simulink library "ASEToolBox"  (R2025b)
settings: Solver=ode45  StartTime=0.0  StopTime=10.0  RelTol=1e-3  EnableMultiTasking=on
values from neighbouring files (symbols this model uses):
  dt = get_param(gcbh, 'g_output_datatype')    [maskSysComCallbacks_Receive.m]    (also in maskSysComCallbacks_Send.m = get_param(gcbh, 'g_input_datatype'))
undefined symbols (not defined in the file or in its folder): dCx, dCy, dCz, DiscIntNeverNeededParam, Discrete, dmassX, dmassY, dmassZ, dMx, dMy, dMz, dp, dp0, dp1, dp2, dp3, dspblkCoreblockFVToolHelper, gcbh, lmd_high, lmd_low, magnitude, Newton, p0, p1, p2, p3, p4, phi0, phi000, phi1, phi2, phi3, phi4, r1, r2, r3, r4, Raphson, theta0, theta1, theta2, theta3, theta4, Time, u0, u1, u2, u3, v0, v0_max, v0_min, v1, v111, v2, v222, v3, v333, v4, W1, w1 ... (+4)
libraries: simulink x38, etargetslib x28, simulink_extras x5, slpidlib x2, ctrlSharedLib x2, aerolibatmos2 x1, aerolibconvert2 x1, aerolibtransform2 x1, sharedtransform x1, dspstat3 x1, dspsolvers x1
(part 5 of 6)

== system ASEToolBox/Subsystem/GNC_EKF/GPS_Data_Process/heading_GPS ==
  Vned : Inport
  Atan2 : Trigonometry  Operator=atan2
  Compare To Constant : simulink/Logic and Bit Operations/Compare To Constant  relop=>  const=0.8  OutDataTypeStr=boolean
  Data Type Conversion : DataTypeConversion  OutDataTypeStr=double  SaturateOnIntegerOverflow=off  RndMeth=Floor
  Math Function : Math  Operator=magnitude^2  SignedPower=on
  Moving Average1 : dspstat3/Moving Average  Commented=on  Method=Sliding window  ForgettingFactorPort=off  SpecifyWindowLength=on  WindowLength=10  OverlapLength=9  AllowArbitraryInputLength=off  ForgettingFactor=0.9  SimulateUsing=Code generation
  Rate Transition : RateTransition  OutPortSampleTime=1
  Scope : Scope  NumInputPorts=2
      settings: ActiveDisplayYMinimum=-3.92587  ActiveDisplayYMaximum=3.91959  DataLoggingVariableName=ScopeData11
  Scope1 : Scope
      settings: ActiveDisplayYMinimum=-0.125  ActiveDisplayYMaximum=1.125  DataLoggingVariableName=ScopeData14
  Selector2 : Selector  InputPortWidth=3  IndexOptions=Index vector (dialog)  Indices=[2]  OutputSizes=1
  Selector3 : Selector  InputPortWidth=3  IndexOptions=Index vector (dialog)  Indices=[1]  OutputSizes=1
  Selector4 : Selector  InputPortWidth=3  IndexOptions=Index vector (dialog)  Indices=[1 2]  OutputSizes=1
  Sqrt : Sqrt
  Sum of Elements : Sum  Inputs=+
  heading_GPS_rad : Outport
  heading_GPS_valid : Outport  Port=2
  wires:
  Selector2/1 -> Atan2/1
  Math Function/1 -> Sum of Elements/1
  Vned/1 -> Selector2/1, Selector4/1, Selector3/1
  Selector3/1 -> Atan2/2
  Sum of Elements/1 -> Sqrt/1
  Selector4/1 -> Math Function/1
  Sqrt/1 -> Data Type Conversion/1
  Compare To Constant/1 -> Scope1/1, heading_GPS_valid/1
  Rate Transition/1 -> Scope/1, Scope/2, heading_GPS_rad/1
  Atan2/1 -> Rate Transition/1
  Data Type Conversion/1 -> Compare To Constant/1

== system ASEToolBox/Subsystem/GNC_EKF/Translation_estimate/Subsystem ==
  vxy : Inport
  pxy_GPS : Inport  Port=2
  GPSv_enable : Inport  Port=3
  QGC_init : Inport  Port=4
  DOP : Inport  Port=5
  Add : Sum  Inputs=+-
  Add1 : Sum  Inputs=++-
  Compare To Constant : simulink/Logic and Bit Operations/Compare To Constant  relop=<=  const=3  OutDataTypeStr=boolean
  Delay : Delay  DelayLength=1  InitialCondition=[0;0;]  ExternalReset=Rising
      settings: InputPortMap=u0,r5
  Detect Change : simulink/Logic and Bit Operations/Detect Change  vinit=0  OutDataTypeStr=boolean
  Gain : Gain  Gain=0.002
  Kalman Filter : ctrlSharedLib/Kalman Filter  TimeDomain=Discrete-Time  UseCurrentEstimator=on  ModelSource=Individual A, B, C, D matrices  ModelSourceVariable=ss(0.95,1,1,0,1)  A=[0.1,0;0,0.1]  B=eye(2)  C=eye(2)  D=0  NumberOfStates=1  NumberOfInputs=1  NumberOfOutputs=1  InitialEstimateSource=Dialog  X0=0  P0=10  UseK=off  UseGH=off  NumberOfProcessNoiseInputs=1  G=1  TimeInvariantG=on  H=0  TimeInvariantH=on  Q=diag([0.1;0.1])  TimeInvariantQ=on  R=diag([0.8;0.8])  TimeInvariantR=on  N=0  TimeInvariantN=on  AddInputPort=off  AddEnablePort=on  ExternalReset=Rising  OutputEstimatedY=off  OutputP=off  Ts=-1
  Logical Operator : Logic  AllPortsSameDT=off  OutDataTypeStr=boolean
  Memory : Memory
  Product : Product  OutDataTypeStr=double
  QGC_init1 : InportShadow  Port=4
  Rate Transition1 : RateTransition  OutPortSampleTime=0.002
  Rate Transition2 : RateTransition  OutPortSampleTime=0.002
  Rate Transition3 : RateTransition  OutPortSampleTime=0.002
  Scope7 : Scope
      settings: ActiveDisplayYMinimum=-0.125  ActiveDisplayYMaximum=1.125
  Selector : Selector  InputPortWidth=2  IndexOptions=Index vector (dialog)  Indices=[1]  OutputSizes=1
  pxy_est : Outport
  wires:
  Gain/1 -> Add1/1
  Delay/1 -> Add1/2
  Kalman Filter/1 -> Product/1
  pxy_GPS/1 -> Selector/1, Add/2
  Selector/1 -> Detect Change/1
  Product/1 -> Memory/1
  Logical Operator/1 -> Product/2, Rate Transition2/1
  Rate Transition2/1 -> Scope7/1, Kalman Filter/2
  Rate Transition1/1 -> Kalman Filter/1
  Memory/1 -> Add1/3
  Add/1 -> Rate Transition1/1
  vxy/1 -> Gain/1
  Add1/1 -> Add/1, Delay/1, pxy_est/1
  QGC_init/1 -> Rate Transition3/1
  Rate Transition3/1 -> Kalman Filter/3
  DOP/1 -> Compare To Constant/1
  Compare To Constant/1 -> Logical Operator/2
  QGC_init1/1 -> Delay/2
  GPSv_enable/1 -> Logical Operator/1

== system ASEToolBox/Subsystem/GNC_EKF/Translation_estimate/Subsystem2 ==
  axy : Inport
  vxy_GPS : Inport  Port=2
  QGC_init : Inport  Port=3
  DOP : Inport  Port=4
  Add : Sum  Inputs=+-
  Add1 : Sum  Inputs=++-
  Compare To Constant : simulink/Logic and Bit Operations/Compare To Constant  relop=<=  const=3  OutDataTypeStr=boolean
  Delay : Delay  DelayLength=1  ExternalReset=Rising
      settings: InputPortMap=u0,r5
  Detect Change : simulink/Logic and Bit Operations/Detect Change  vinit=0  OutDataTypeStr=boolean
  Gain : Gain  Gain=0.002
  Kalman Filter : ctrlSharedLib/Kalman Filter  TimeDomain=Discrete-Time  UseCurrentEstimator=on  ModelSource=Individual A, B, C, D matrices  ModelSourceVariable=ss(0.95,1,1,0,1)  A=[0.6,0;0,0.6]  B=eye(2)  C=eye(2)  D=0  NumberOfStates=1  NumberOfInputs=1  NumberOfOutputs=1  InitialEstimateSource=Dialog  X0=0  P0=10  UseK=off  UseGH=off  NumberOfProcessNoiseInputs=1  G=1  TimeInvariantG=on  H=0  TimeInvariantH=on  Q=diag([0.1;0.1])  TimeInvariantQ=on  R=diag([0.6;0.6])  TimeInvariantR=on  N=0  TimeInvariantN=on  AddInputPort=off  AddEnablePort=on  ExternalReset=Rising  OutputEstimatedY=off  OutputP=off  Ts=-1
  Logical Operator : Logic  AllPortsSameDT=off  OutDataTypeStr=boolean
  Memory : Memory
  Product : Product  OutDataTypeStr=double
  Rate Transition1 : RateTransition  OutPortSampleTime=0.002
  Rate Transition2 : RateTransition  OutPortSampleTime=0.002
  Rate Transition3 : RateTransition  OutPortSampleTime=0.002
  Scope : Scope  NumInputPorts=2
      settings: ActiveDisplayYMinimum=-13.99764  ActiveDisplayYMaximum=33.23237
  Scope7 : Scope
      settings: ActiveDisplayYMinimum=-0.125  ActiveDisplayYMaximum=1.125
  Selector : Selector  InputPortWidth=2  IndexOptions=Index vector (dialog)  Indices=[1]  OutputSizes=1
  vxy_est : Outport
  GPSv_enable : Outport  Port=2
  wires:
  Compare To Constant/1 -> Logical Operator/2
  DOP/1 -> Compare To Constant/1
  Detect Change/1 -> Logical Operator/1
  Rate Transition3/1 -> Kalman Filter/3
  QGC_init/1 -> Delay/2, Rate Transition3/1
  Add1/1 -> Delay/1, vxy_est/1, Scope/1, Add/1
  Add/1 -> Rate Transition1/1
  Memory/1 -> Add1/3
  Rate Transition1/1 -> Kalman Filter/1
  Rate Transition2/1 -> Scope7/1, Kalman Filter/2
  Logical Operator/1 -> GPSv_enable/1, Rate Transition2/1, Product/2
  Product/1 -> Memory/1
  Selector/1 -> Detect Change/1
  vxy_GPS/1 -> Selector/1, Add/2, Scope/2
  Kalman Filter/1 -> Product/1
  Gain/1 -> Add1/1
  axy/1 -> Gain/1
  Delay/1 -> Add1/2

== system ASEToolBox/Subsystem/GNC_EKF/Translation_estimate/V_Horizontal_estimation1 ==
  note: 0530改：
      | 加入GPStype限制
  An : Inport
  vn_gps : Inport  Port=2
  ve_gps : Inport  Port=3
  fixtype_gps : Inport  Port=4
  QGC_init : Inport  Port=5
  Add : Sum  Inputs=+-
  Compare To Constant : simulink/Logic and Bit Operations/Compare To Constant  relop=>=  const=3  OutDataTypeStr=boolean
  Delay : Delay  DelayLength=1
  Detect Change : simulink/Logic and Bit Operations/Detect Change  vinit=0  OutDataTypeStr=boolean
  Integrator_V_Horizontal : Subsystem
  Logical Operator : Logic  AllPortsSameDT=off  OutDataTypeStr=boolean
  Mux : Mux  Inputs=2
  Rxy_kalman filter1 : Subsystem  mask{F=diag([-0.1,-0.1,-0.002,-0.002]), H=[1,0,-1,0;0,1,0,-1], Q=diag([1,1,0.1,0.1]), R=diag([0.001,0.001]), P0=diag([0.8,0.8,0.2,0.2])}
      mask prompts: F "状态转移矩阵：F"; H "观测转移矩阵：H"; Q "预测噪声协方差矩阵：Q"; R "量测噪声协方差矩阵：R"; P0 "初始协方差矩阵：P0"
      mask DialogControl DescTextVar Prompt: Kalman Filter
  Scope : Scope  NumInputPorts=2
      settings: ActiveDisplayYMinimum=-0.21744  ActiveDisplayYMaximum=0.36084  DataLoggingVariableName=ScopeData16
  Scope1 : Scope
      settings: ActiveDisplayYMinimum=0.9  ActiveDisplayYMaximum=1.1
  Selector : Selector  InputPortWidth=4  IndexOptions=Index vector (dialog)  Indices=[1 2]  OutputSizes=1
  vxy_estimout : Outport
  GPS_v_enable : Outport  Port=2
  wires:
  QGC_init/1 -> Integrator_V_Horizontal/3(QGC_init)
  Delay/1 -> Selector/1, Rxy_kalman filter1/1(X)
  Selector/1 -> Integrator_V_Horizontal/2(dv)
  vn_gps/1 -> Integrator_V_Horizontal/4(vn_gps), Mux/1, Detect Change/1
  Mux/1 -> Scope/2, Add/2
  ve_gps/1 -> Integrator_V_Horizontal/5(ve_gps), Mux/2
  Rxy_kalman filter1/1(XOut) -> Delay/1
  Integrator_V_Horizontal/1(V_n&e) -> Add/1, vxy_estimout/1, Scope/1
  Add/1 -> Rxy_kalman filter1/2(Z)
  An/1 -> Integrator_V_Horizontal/1(An)
  fixtype_gps/1 -> Compare To Constant/1
  Detect Change/1 -> Logical Operator/1
  Compare To Constant/1 -> Logical Operator/2, Scope1/1, GPS_v_enable/1, Rxy_kalman filter1/3(Enable), Integrator_V_Horizontal/6(GPSenable)

== system ASEToolBox/Subsystem/GNC_EKF/Translation_estimate/translate to N ==
  Cbn : Inport
  accl_ned : Inport  Port=2
  Product : Product  Multiplication=Matrix(*)
  Selector : Selector  InputPortWidth=3  IndexOptions=Index vector (dialog)  Indices=[1 2]  OutputSizes=1
  accel_Horizontal_predict : Outport
  wires:
  Selector/1 -> accel_Horizontal_predict/1
  Product/1 -> Selector/1
  Cbn/1 -> Product/1
  accl_ned/1 -> Product/2

== system ASEToolBox/Aerocraft Model/ACE Equation of 6DOF's Motion/ACE Centroid Motion/231 Motion Subsystem/Deal with zero1 ==
  In1 : Inport
  Constant : Constant  Value=0
  Constant1 : Constant  Value=0.000001
  Relational Operator : RelationalOperator  Operator=~=
  Switch : Switch  Threshold=0.0001
  Out1 : Outport
  wires:
  In1/1 -> Relational Operator/1, Switch/1
  Switch/1 -> Out1/1
  Constant1/1 -> Switch/3
  Relational Operator/1 -> Switch/2
  Constant/1 -> Relational Operator/2

== system ASEToolBox/Aerocraft Model/ACE Equation of 6DOF's Motion/ACE Centroid Motion/231 Motion Subsystem/Deal with zero2 ==
  In1 : Inport
  Constant : Constant  Value=0
  Constant1 : Constant  Value=0.000001
  Relational Operator : RelationalOperator  Operator=~=
  Switch : Switch  Threshold=0.0001
  Out1 : Outport
  wires:
  Constant/1 -> Relational Operator/2
  Relational Operator/1 -> Switch/2
  Constant1/1 -> Switch/3
  Switch/1 -> Out1/1
  In1/1 -> Switch/1, Relational Operator/1

== system ASEToolBox/Aerocraft Model/ACE Equation of 6DOF's Motion/ACE Centroid Motion/231 Motion Subsystem/Deal with zero3 ==
  In1 : Inport
  Constant : Constant  Value=0
  Constant1 : Constant  Value=0.000001
  Relational Operator : RelationalOperator  Operator=~=
  Switch : Switch  Threshold=0.0001
  Out1 : Outport
  wires:
  Constant/1 -> Relational Operator/2
  Relational Operator/1 -> Switch/2
  Constant1/1 -> Switch/3
  Switch/1 -> Out1/1
  In1/1 -> Switch/1, Relational Operator/1

== system ASEToolBox/Aerocraft Model/ACE Equation of 6DOF's Motion/ACE Rotation Motion/Attitude Dynamic /Omega_Tx1 Subsystem ==
  note: d( w_x ) = [M_x + (I_y-I_z)*w_y*w_z)] / I_x
      | .
  note: rad/s
  Wxyz : Inport
  Ixyz : Inport  Port=2
  Mxyz : Inport  Port=3
  Deal with zero : Subsystem
  Demux6 : Demux  Outputs=3
  Discrete-Time Integrator : DiscreteIntegrator  SampleTime=-1  ICPrevOutput=DiscIntNeverNeededParam  ICPrevScaledInput=DiscIntNeverNeededParam
  Integrator1 : Integrator  Commented=on
  Product4 : Product  Inputs=***  InputSameDT=on  SaturateOnIntegerOverflow=on  OutDataTypeStr=Inherit: Same as first input
  Product6 : Product  Inputs=/*  InputSameDT=on  SaturateOnIntegerOverflow=on  OutDataTypeStr=Inherit: Same as first input
  Selector1 : Selector  InputPortWidth=3  IndexOptions=Index vector (dialog)  Indices=2  OutputSizes=1
  Selector2 : Selector  InputPortWidth=3  IndexOptions=Index vector (dialog)  Indices=1  OutputSizes=1
  Selector3 : Selector  InputPortWidth=3  IndexOptions=Index vector (dialog)  Indices=3  OutputSizes=1
  Sum1 : Sum  Inputs=+-  InputSameDT=on  SaturateOnIntegerOverflow=on  OutDataTypeStr=Inherit: Same as first input
  Sum6 : Sum  InputSameDT=on  SaturateOnIntegerOverflow=on  OutDataTypeStr=Inherit: Same as first input
  Wx : Outport
  wires:
  Discrete-Time Integrator/1 -> Wx/1
  Mxyz/1 -> Selector2/1
  Product6/1 -> Discrete-Time Integrator/1
  Wxyz/1 -> Selector1/1, Selector3/1
  Sum1/1 -> Product4/1
  Selector1/1 -> Product4/2  "Omega_y"
  Selector3/1 -> Product4/3  "Omega_z"
  Product4/1 -> Sum6/1
  Selector2/1 -> Sum6/2  "Mx"
  Sum6/1 -> Product6/2
  Ixyz/1 -> Demux6/1
  Demux6/2 -> Sum1/1
  Demux6/3 -> Sum1/2
  Demux6/1 -> Deal with zero/1(In1)
  Deal with zero/1(Out1) -> Product6/1

== system ASEToolBox/Aerocraft Model/ACE Equation of 6DOF's Motion/ACE Rotation Motion/Attitude Dynamic /Omega_Tx1 Subsystem1 ==
  note: rad/s
  note: d( w_y ) = M_y + (I_z-I_x)*w_x*w_z)
      |
      |  / I_y
      | .
  Wxyz : Inport
  Ixyz : Inport  Port=2
  Mxyz : Inport  Port=3
  Deal with zero : Subsystem
  Demux6 : Demux  Outputs=3
  Discrete-Time Integrator : DiscreteIntegrator  SampleTime=-1  ICPrevOutput=DiscIntNeverNeededParam  ICPrevScaledInput=DiscIntNeverNeededParam
  Integrator1 : Integrator  Commented=on
  Product4 : Product  Inputs=***  InputSameDT=on  SaturateOnIntegerOverflow=on  OutDataTypeStr=Inherit: Same as first input
  Product6 : Product  Inputs=/*  InputSameDT=on  SaturateOnIntegerOverflow=on  OutDataTypeStr=Inherit: Same as first input
  Selector1 : Selector  InputPortWidth=3  IndexOptions=Index vector (dialog)  Indices=1  OutputSizes=1
  Selector2 : Selector  InputPortWidth=3  IndexOptions=Index vector (dialog)  Indices=2  OutputSizes=1
  Selector3 : Selector  InputPortWidth=3  IndexOptions=Index vector (dialog)  Indices=3  OutputSizes=1
  Sum1 : Sum  Inputs=-+  InputSameDT=on  SaturateOnIntegerOverflow=on  OutDataTypeStr=Inherit: Same as first input
  Sum6 : Sum  InputSameDT=on  SaturateOnIntegerOverflow=on  OutDataTypeStr=Inherit: Same as first input
  Wy : Outport
  wires:
  Discrete-Time Integrator/1 -> Wy/1
  Deal with zero/1(Out1) -> Product6/1
  Ixyz/1 -> Demux6/1
  Sum6/1 -> Product6/2
  Selector2/1 -> Sum6/2  "My"
  Product4/1 -> Sum6/1
  Selector3/1 -> Product4/3  "Omega_z"
  Selector1/1 -> Product4/2  "Omega_x"
  Sum1/1 -> Product4/1
  Wxyz/1 -> Selector3/1, Selector1/1
  Product6/1 -> Discrete-Time Integrator/1
  Mxyz/1 -> Selector2/1
  Demux6/3 -> Sum1/2
  Demux6/1 -> Sum1/1
  Demux6/2 -> Deal with zero/1(In1)

== system ASEToolBox/Aerocraft Model/ACE Equation of 6DOF's Motion/ACE Rotation Motion/Attitude Dynamic /Omega_Tx1 Subsystem2 ==
  note: d( w_z ) = M_z + (I_x-I_y)*w_x*w_y)
      |
      |  / I_z
      | .
  note: rad/s
  Wxyz : Inport
  Ixyz : Inport  Port=2
  Mxyz : Inport  Port=3
  Deal with zero : Subsystem
  Demux6 : Demux  Outputs=3
  Discrete-Time Integrator : DiscreteIntegrator  SampleTime=-1  ICPrevOutput=DiscIntNeverNeededParam  ICPrevScaledInput=DiscIntNeverNeededParam
  Integrator1 : Integrator  Commented=on
  Product4 : Product  Inputs=***  InputSameDT=on  SaturateOnIntegerOverflow=on  OutDataTypeStr=Inherit: Same as first input
  Product6 : Product  Inputs=/*  InputSameDT=on  SaturateOnIntegerOverflow=on  OutDataTypeStr=Inherit: Same as first input
  Selector1 : Selector  InputPortWidth=3  IndexOptions=Index vector (dialog)  Indices=1  OutputSizes=1
  Selector2 : Selector  InputPortWidth=3  IndexOptions=Index vector (dialog)  Indices=3  OutputSizes=1
  Selector3 : Selector  InputPortWidth=3  IndexOptions=Index vector (dialog)  Indices=2  OutputSizes=1
  Sum1 : Sum  Inputs=+-  InputSameDT=on  SaturateOnIntegerOverflow=on  OutDataTypeStr=Inherit: Same as first input
  Sum6 : Sum  InputSameDT=on  SaturateOnIntegerOverflow=on  OutDataTypeStr=Inherit: Same as first input
  Wz : Outport
  wires:
  Discrete-Time Integrator/1 -> Wz/1
  Mxyz/1 -> Selector2/1
  Product6/1 -> Discrete-Time Integrator/1
  Wxyz/1 -> Selector1/1, Selector3/1
  Sum1/1 -> Product4/1
  Selector1/1 -> Product4/2  "Omega_x"
  Selector3/1 -> Product4/3  "Omega_y"
  Product4/1 -> Sum6/1
  Selector2/1 -> Sum6/2  "Mz"
  Sum6/1 -> Product6/2
  Ixyz/1 -> Demux6/1
  Deal with zero/1(Out1) -> Product6/1
  Demux6/1 -> Sum1/1
  Demux6/2 -> Sum1/2
  Demux6/3 -> Deal with zero/1(In1)

== system ASEToolBox/Aerocraft Model/ACE Equation of 6DOF's Motion/ACE Rotation Motion/calculate Eular 231/gam Subsystem ==
  note: d \gamma = W_x - tan \phi * ( W_y * cos \gamma - W_z * sin \gamma )
  Eular : Inport
  Wxyz : Inport  Port=2
  Eular0 : Inport  Port=3
  Demux6 : Demux  Outputs=3
  Discrete-Time Integrator : DiscreteIntegrator  InitialConditionSource=external  SampleTime=-1  ICPrevOutput=DiscIntNeverNeededParam  ICPrevScaledInput=DiscIntNeverNeededParam
  Integrator1 : Integrator  Commented=on  InitialConditionSource=external
  Product10 : Product  RndMeth=Zero
  Product8 : Product  Inputs=**  InputSameDT=on  SaturateOnIntegerOverflow=on  OutDataTypeStr=Inherit: Same as first input
  Product9 : Product  RndMeth=Zero
  Selector1 : Selector  InputPortWidth=3  IndexOptions=Index vector (dialog)  Indices=3  OutputSizes=1
  Selector2 : Selector  InputPortWidth=3  IndexOptions=Index vector (dialog)  Indices=3  OutputSizes=1
  Selector3 : Selector  InputPortWidth=3  IndexOptions=Index vector (dialog)  Indices=2  OutputSizes=1
  Selector5 : Selector  InputPortWidth=3  IndexOptions=Index vector (dialog)  Indices=1  OutputSizes=1
  Sum1 : Sum  Inputs=-+  InputSameDT=on  SaturateOnIntegerOverflow=on  OutDataTypeStr=Inherit: Same as first input
  Sum6 : Sum  Inputs=-+  InputSameDT=on  SaturateOnIntegerOverflow=on  OutDataTypeStr=Inherit: Same as first input
  Terminator : Terminator
  Trigonometric Function4 : Trigonometry  Operator=cos
  Trigonometric Function5 : Trigonometry
  Trigonometric Function6 : Trigonometry  Operator=tan
  gam : Outport
  wires:
  Sum1/1 -> Discrete-Time Integrator/1
  Product8/1 -> Sum1/1
  Selector1/1 -> Discrete-Time Integrator/2
  Selector5/1 -> Sum1/2
  Eular0/1 -> Selector1/1
  Eular/1 -> Demux6/1
  Demux6/3 -> Trigonometric Function5/1, Trigonometric Function4/1  "gam"
  Discrete-Time Integrator/1 -> gam/1
  Trigonometric Function6/1 -> Product8/2
  Sum6/1 -> Product8/1
  Product9/1 -> Sum6/2
  Product10/1 -> Sum6/1
  Trigonometric Function5/1 -> Product10/1
  Selector2/1 -> Product10/2
  Trigonometric Function4/1 -> Product9/2
  Selector3/1 -> Product9/1
  Wxyz/1 -> Selector5/1, Selector2/1, Selector3/1
  Demux6/2 -> Terminator/1  "psi"
  Demux6/1 -> Trigonometric Function6/1  "phi"

== system ASEToolBox/Aerocraft Model/ACE Equation of 6DOF's Motion/ACE Rotation Motion/calculate Eular 231/phi Subsystem ==
  note: d \phi = W_y * sin \gamma + W_z * cos \gamma
  Eular : Inport
  Wxyz : Inport  Port=2
  Eular0 : Inport  Port=3
  Demux6 : Demux  Outputs=3
  Discrete-Time Integrator : DiscreteIntegrator  InitialConditionSource=external  SampleTime=-1  ICPrevOutput=DiscIntNeverNeededParam  ICPrevScaledInput=DiscIntNeverNeededParam
  Integrator1 : Integrator  Commented=on  InitialConditionSource=external
  Product10 : Product  RndMeth=Zero
  Product9 : Product  RndMeth=Zero
  Selector1 : Selector  InputPortWidth=3  IndexOptions=Index vector (dialog)  Indices=1  OutputSizes=1
  Selector2 : Selector  InputPortWidth=3  IndexOptions=Index vector (dialog)  Indices=3  OutputSizes=1
  Selector3 : Selector  InputPortWidth=3  IndexOptions=Index vector (dialog)  Indices=2  OutputSizes=1
  Sum6 : Sum  InputSameDT=on  SaturateOnIntegerOverflow=on  OutDataTypeStr=Inherit: Same as first input
  Terminator : Terminator
  Terminator1 : Terminator
  Trigonometric Function4 : Trigonometry
  Trigonometric Function5 : Trigonometry  Operator=cos
  phi : Outport
  wires:
  Selector1/1 -> Discrete-Time Integrator/2
  Eular0/1 -> Selector1/1
  Demux6/1 -> Terminator/1  "phi"
  Eular/1 -> Demux6/1
  Demux6/3 -> Trigonometric Function5/1, Trigonometric Function4/1  "gam"
  Discrete-Time Integrator/1 -> phi/1
  Product9/1 -> Sum6/2
  Product10/1 -> Sum6/1
  Trigonometric Function5/1 -> Product10/1
  Selector2/1 -> Product10/2
  Trigonometric Function4/1 -> Product9/2
  Selector3/1 -> Product9/1
  Wxyz/1 -> Selector2/1, Selector3/1
  Demux6/2 -> Terminator1/1  "psi"
  Sum6/1 -> Discrete-Time Integrator/1

== system ASEToolBox/Aerocraft Model/ACE Equation of 6DOF's Motion/ACE Rotation Motion/calculate Eular 231/psi Subsystem ==
  note: d \psi = (W_y * cos \gamma - W_z * sin \gamma ) / cos \phi
  Eular : Inport
  Wxyz : Inport  Port=2
  Eular0 : Inport  Port=3
  Deal with zero1 : Subsystem
  Demux6 : Demux  Outputs=3
  Discrete-Time Integrator : DiscreteIntegrator  InitialConditionSource=external  SampleTime=-1  ICPrevOutput=DiscIntNeverNeededParam  ICPrevScaledInput=DiscIntNeverNeededParam
  Integrator1 : Integrator  Commented=on  InitialConditionSource=external
  Product10 : Product  RndMeth=Zero
  Product8 : Product  Inputs=*/  InputSameDT=on  SaturateOnIntegerOverflow=on  OutDataTypeStr=Inherit: Same as first input
  Product9 : Product  RndMeth=Zero
  Selector1 : Selector  InputPortWidth=3  IndexOptions=Index vector (dialog)  Indices=2  OutputSizes=1
  Selector2 : Selector  InputPortWidth=3  IndexOptions=Index vector (dialog)  Indices=3  OutputSizes=1
  Selector3 : Selector  InputPortWidth=3  IndexOptions=Index vector (dialog)  Indices=2  OutputSizes=1
  Sum6 : Sum  Inputs=-+  InputSameDT=on  SaturateOnIntegerOverflow=on  OutDataTypeStr=Inherit: Same as first input
  Terminator1 : Terminator
  Trigonometric Function1 : Trigonometry  Operator=cos
  Trigonometric Function4 : Trigonometry  Operator=cos
  Trigonometric Function5 : Trigonometry
  psi : Outport
  wires:
  Demux6/2 -> Terminator1/1  "psi"
  Wxyz/1 -> Selector3/1, Selector2/1
  Selector3/1 -> Product9/1
  Trigonometric Function4/1 -> Product9/2
  Selector2/1 -> Product10/2
  Trigonometric Function5/1 -> Product10/1
  Product10/1 -> Sum6/1
  Product9/1 -> Sum6/2
  Discrete-Time Integrator/1 -> psi/1
  Demux6/3 -> Trigonometric Function5/1, Trigonometric Function4/1  "gam"
  Eular/1 -> Demux6/1
  Eular0/1 -> Selector1/1
  Selector1/1 -> Discrete-Time Integrator/2
  Sum6/1 -> Product8/1
  Trigonometric Function1/1 -> Deal with zero1/1(In1)
  Demux6/1 -> Trigonometric Function1/1  "phi"
  Product8/1 -> Discrete-Time Integrator/1
  Deal with zero1/1(Out1) -> Product8/2

== system ASEToolBox/Aerocraft Model/ACE Equation of 6DOF's Motion/Aero Force & Moment/ACE Aerodynamic for 6DOF/CL Subsystem ==
  alpha : Inport
  Ma : Inport  Port=2
  DeltZ : Inport  Port=3
  Add : Sum
  CL0 : Lookup2D  RowIndex=[-2,-1,0.5,1:10]  ColumnIndex=[0.3:0.1:0.8]  Table=|  SaturateOnIntegerOverflow=off  InputSameDT=off
      | [-0.8551	-0.8635	-0.8752	-0.8919	-0.914	-0.9479
      | -0.4232	-0.4273	-0.4332	-0.4415	-0.4525	-0.4695
      | 0.2105	0.2126	0.2155	0.2196	0.2251	0.2336
      | 0.4232	0.4273	0.4332	0.4415	0.4525	0.4695
      | 0.8551	0.8635	0.8752	0.8919	0.914	0.9479
      | 1.2956	1.3082	1.3258	1.351	1.3842	1.4353
      | 1.7443	1.7612	1.7848	1.8186	1.863	1.9315
      | 2.201	2.2223	2.2519	2.2944	2.3504	2.4364
      | 2.6653	2.691	2.7269	2.7783	2.846	2.95
      | 3.1369	3.1673	3.2096	3.2701	3.3498	3.4721
      | 3.6156	3.6507	3.6996	3.7695	3.8615	4.0026
      | 4.101	4.1411	4.1967	4.2764	4.381	4.5414
      | 4.593	4.6381	4.7008	4.7905	4.9082	5.0886
      | ]
  CLDeltZ : Lookup2D  RowIndex=|  ColumnIndex=|  Table=|  SaturateOnIntegerOverflow=off  InputSameDT=off
      RowIndex=|
      | [-2
      | -1
      | 0.5
      | 1
      | 2
      | 3
      | 4
      | 5
      | 6
      | 7
      | 8
      | 9
      | 10
      | ]
      Table=|
      | [0.0513	0.0522	0.0532	0.0541	0.0541	0.0541
      | 0.0513	0.0523	0.0532	0.0542	0.0542	0.0542
      | 0.0514	0.0523	0.0533	0.0542	0.0542	0.0542
      | 0.0513	0.0523	0.0532	0.0542	0.0542	0.0542
      | 0.0513	0.0522	0.0532	0.0541	0.0541	0.0541
      | 0.0512	0.0521	0.0531	0.054	0.054	0.054
      | 0.0511	0.052	0.053	0.0539	0.0539	0.0539
      | 0.0509	0.0518	0.0528	0.0537	0.0537	0.0537
      | 0.0507	0.0516	0.0526	0.0535	0.0535	0.0535
      | 0.0505	0.0514	0.0523	0.0533	0.0533	0.0533
      | 0.0502	0.0511	0.0521	0.053	0.053	0.053
      | 0.0499	0.0508	0.0517	0.0527	0.0527	0.0527
      | 0.0496	0.0505	0.0514	0.0523	0.0523	0.0523
      | ]
      ColumnIndex=|
      | [0.3	0.4	0.5	0.6	0.7	0.8
      | ]
  Divide1 : Product  Inputs=**
  CL : Outport
  wires:
  DeltZ/1 -> Divide1/1
  Ma/1 -> CLDeltZ/2, CL0/2
  alpha/1 -> CLDeltZ/1, CL0/1
  CLDeltZ/1 -> Divide1/2
  CL0/1 -> Add/1
  Divide1/1 -> Add/2
  Add/1 -> CL/1

== system ASEToolBox/Aerocraft Model/ACE Equation of 6DOF's Motion/Aero Force & Moment/ACE Aerodynamic for 6DOF/CZ Subsystem ==
  beta : Inport
  alpha : Inport  Port=2
  Ma : Inport  Port=3
  CZBETA : Lookup2D  RowIndex=|  ColumnIndex=|  Table=|  SaturateOnIntegerOverflow=off  InputSameDT=off
      RowIndex=|
      | [-2
      | -1
      | 0.5
      | 1
      | 2
      | 3
      | 4
      | 5
      | 6
      | 7
      | 8
      | 9
      | 10
      | ]
      Table=|
      | [-0.3754	-0.3669	-0.3551	-0.3384	-0.3165	-0.2829
      | -0.3758	-0.3672	-0.3555	-0.3387	-0.3168	-0.2831
      | -0.3759	-0.3673	-0.3555	-0.3388	-0.3169	-0.2832
      | -0.3758	-0.3672	-0.3555	-0.3387	-0.3168	-0.2831
      | -0.3754	-0.3669	-0.3551	-0.3384	-0.3165	-0.2829
      | -0.3748	-0.3663	-0.3545	-0.3379	-0.316	-0.2824
      | -0.374	-0.3655	-0.3538	-0.3371	-0.3153	-0.2818
      | -0.3729	-0.3644	-0.3527	-0.3361	-0.3144	-0.281
      | -0.3716	-0.3631	-0.3515	-0.335	-0.3133	-0.2801
      | -0.37	-0.3616	-0.35	-0.3336	-0.312	-0.279
      | -0.3682	-0.3599	-0.3484	-0.332	-0.3106	-0.2777
      | -0.3662	-0.3579	-0.3465	-0.3302	-0.3089	-0.2762
      | -0.364	-0.3557	-0.3444	-0.3282	-0.3071	-0.2746
      | ]
      ColumnIndex=|
      | [0.3	0.4	0.5	0.6	0.7	0.8
      | ]
  Divide : Product  Inputs=**
  CZ : Outport
  wires:
  Ma/1 -> CZBETA/2
  alpha/1 -> CZBETA/1
  Divide/1 -> CZ/1
  CZBETA/1 -> Divide/2
  beta/1 -> Divide/1

== system ASEToolBox/Aerocraft Model/ACE Equation of 6DOF's Motion/Aero Force & Moment/ACE Aerodynamic for 6DOF/Mx Subsystem ==
  Beta : Inport
  Ma : Inport  Port=2
  alpha : Inport  Port=3
  DeltX : Inport  Port=4
  WX : Inport  Port=5
  WY : Inport  Port=6
  Add1 : Sum  Inputs=++++
  Divide{,2..4} (4 alike) : Product  Inputs=**
  MXBETA : Lookup2D  RowIndex=|  ColumnIndex=|  Table=|  SaturateOnIntegerOverflow=off  InputSameDT=off
      RowIndex=|
      | [-2
      | -1
      | 0.5
      | 1
      | 2
      | 3
      | 4
      | 5
      | 6
      | 7
      | 8
      | 9
      | 10
      | ]
      Table=|
      | [-0.0008	-0.0009	-0.0009	-0.0011	-0.0012	-0.0015
      | -0.0024	-0.0024	-0.0025	-0.0025	-0.0026	-0.0027
      | -0.0048	-0.0048	-0.0048	-0.0047	-0.0047	-0.0046
      | -0.0056	-0.0056	-0.0055	-0.0055	-0.0054	-0.0053
      | -0.0072	-0.0072	-0.0071	-0.0069	-0.0068	-0.0065
      | -0.0088	-0.0087	-0.0086	-0.0084	-0.0082	-0.0078
      | -0.0104	-0.0103	-0.0101	-0.0099	-0.0095	-0.009
      | -0.012	-0.0118	-0.0116	-0.0113	-0.0109	-0.0103
      | -0.0135	-0.0133	-0.0131	-0.0127	-0.0122	-0.0115
      | -0.015	-0.0148	-0.0145	-0.0141	-0.0135	-0.0127
      | -0.0165	-0.0163	-0.0159	-0.0155	-0.0148	-0.0139
      | -0.018	-0.0177	-0.0173	-0.0168	-0.0161	-0.015
      | -0.0194	-0.0191	-0.0187	-0.0181	-0.0174	-0.0162
      | ]
      ColumnIndex=|
      | [0.3	0.4	0.5	0.6	0.7	0.8
      | ]
  MXDeltX : Lookup2D  RowIndex=|  ColumnIndex=|  Table=|  SaturateOnIntegerOverflow=off  InputSameDT=off
      RowIndex=|
      | [-2
      | -1
      | 0.5
      | 1
      | 2
      | 3
      | 4
      | 5
      | 6
      | 7
      | 8
      | 9
      | 10
      | ]
      Table=|
      | [0.0035	0.0036	0.0037	0.0039	0.0042	0.0045
      | 0.0035	0.0036	0.0037	0.0039	0.0042	0.0045
      | 0.0035	0.0036	0.0037	0.0039	0.0042	0.0045
      | 0.0035	0.0036	0.0037	0.0039	0.0042	0.0045
      | 0.0035	0.0036	0.0037	0.0039	0.0042	0.0045
      | 0.0035	0.0036	0.0037	0.0039	0.0042	0.0045
      | 0.0034	0.0035	0.0037	0.0039	0.0042	0.0045
      | 0.0034	0.0035	0.0037	0.0039	0.0042	0.0045
      | 0.0034	0.0035	0.0037	0.0039	0.0042	0.0045
      | 0.0034	0.0035	0.0037	0.0039	0.0042	0.0045
      | 0.0034	0.0035	0.0037	0.0039	0.0041	0.0045
      | 0.0034	0.0035	0.0037	0.0039	0.0041	0.0045
      | 0.0034	0.0035	0.0037	0.0039	0.0041	0.0045
      | ]
      ColumnIndex=|
      | [0.3	0.4	0.5	0.6	0.7	0.8
      | ]
  MXWX : Lookup2D  RowIndex=|  ColumnIndex=|  Table=|  SaturateOnIntegerOverflow=off  InputSameDT=off
      RowIndex=|
      | [-2
      | -1
      | 0.5
      | 1
      | 2
      | 3
      | 4
      | 5
      | 6
      | 7
      | 8
      | 9
      | 10
      | ]
      Table=|
      | [-0.0034	-0.0033	-0.0033	-0.0031	-0.0031	-0.0032
      | -0.0037	-0.0036	-0.0035	-0.0033	-0.0033	-0.0034
      | -0.004	-0.004	-0.0039	-0.0037	-0.0036	-0.0036
      | -0.0041	-0.0041	-0.004	-0.0038	-0.0037	-0.0037
      | -0.0044	-0.0043	-0.0042	-0.0039	-0.0039	-0.0039
      | -0.0045	-0.0045	-0.0044	-0.0041	-0.0041	-0.004
      | -0.0047	-0.0046	-0.0045	-0.0043	-0.0042	-0.0041
      | -0.0048	-0.0047	-0.0046	-0.0044	-0.0043	-0.0042
      | -0.0049	-0.0048	-0.0047	-0.0045	-0.0044	-0.0043
      | -0.005	-0.0049	-0.0048	-0.0045	-0.0045	-0.0044
      | -0.0051	-0.005	-0.0049	-0.0046	-0.0045	-0.0044
      | -0.0051	-0.005	-0.0049	-0.0046	-0.0045	-0.0044
      | -0.0051	-0.005	-0.0049	-0.0046	-0.0045	-0.0044
      | ]
      ColumnIndex=|
      | [0.3	0.4	0.5	0.6	0.7	0.8
      | ]
  MXWY : Lookup2D  RowIndex=|  ColumnIndex=|  Table=|  SaturateOnIntegerOverflow=off  InputSameDT=off
      RowIndex=|
      | [-2
      | -1
      | 0.5
      | 1
      | 2
      | 3
      | 4
      | 5
      | 6
      | 7
      | 8
      | 9
      | 10
      | ]
      Table=|
      | [-0.0152	-0.0148	-0.0143	-0.0135	-0.0125	-0.011
      | -0.0146	-0.0143	-0.0138	-0.013	-0.0121	-0.0106
      | -0.0138	-0.0134	-0.013	-0.0123	-0.0114	-0.01
      | -0.0135	-0.0132	-0.0127	-0.012	-0.0112	-0.0099
      | -0.0129	-0.0126	-0.0122	-0.0115	-0.0107	-0.0095
      | -0.0123	-0.012	-0.0116	-0.011	-0.0103	-0.0091
      | -0.0117	-0.0115	-0.0111	-0.0105	-0.0098	-0.0087
      | -0.0112	-0.0109	-0.0105	-0.01	-0.0093	-0.0083
      | -0.0106	-0.0104	-0.01	-0.0095	-0.0089	-0.0079
      | -0.0101	-0.0098	-0.0095	-0.0091	-0.0085	-0.0076
      | -0.0095	-0.0093	-0.009	-0.0086	-0.008	-0.0072
      | -0.009	-0.0088	-0.0086	-0.0082	-0.0077	-0.0069
      | -0.0086	-0.0084	-0.0081	-0.0078	-0.0073	-0.0066
      | ]
      ColumnIndex=|
      | [0.3	0.4	0.5	0.6	0.7	0.8
      | ]
  Mx : Outport
  wires:
  Beta/1 -> Divide/2
  Ma/1 -> MXBETA/2, MXDeltX/2, MXWX/2, MXWY/2
  alpha/1 -> MXBETA/1, MXDeltX/1, MXWX/1, MXWY/1
  Add1/1 -> Mx/1
  Divide4/1 -> Add1/4
  Divide3/1 -> Add1/3
  Divide2/1 -> Add1/2
  Divide/1 -> Add1/1
  WY/1 -> Divide4/2
  MXWY/1 -> Divide4/1
  WX/1 -> Divide3/2
  MXWX/1 -> Divide3/1
  DeltX/1 -> Divide2/2
  MXDeltX/1 -> Divide2/1
  MXBETA/1 -> Divide/1

== system ASEToolBox/Aerocraft Model/ACE Equation of 6DOF's Motion/Aero Force & Moment/ACE Aerodynamic for 6DOF/My Subsystem ==
  Beta : Inport
  WX : Inport  Port=2
  WY : Inport  Port=3
  Ma : Inport  Port=4
  alpha : Inport  Port=5
  Add2 : Sum  Inputs=+++
  Divide1 : Product  Inputs=**
  Divide2 : Product  Inputs=**
  Divide3 : Product  Inputs=**
  MYBETA : Lookup2D  RowIndex=|  ColumnIndex=|  Table=|  SaturateOnIntegerOverflow=off  InputSameDT=off
      RowIndex=|
      | [-2
      | -1
      | 0.5
      | 1
      | 2
      | 3
      | 4
      | 5
      | 6
      | 7
      | 8
      | 9
      | 10
      | ]
      Table=|
      | [-0.083	-0.0809	-0.078	-0.074	-0.0686	-0.0604
      | -0.0831	-0.081	-0.0781	-0.074	-0.0687	-0.0604
      | -0.083	-0.0809	-0.078	-0.0739	-0.0686	-0.0603
      | -0.0829	-0.0808	-0.078	-0.0739	-0.0685	-0.0603
      | -0.0827	-0.0806	-0.0778	-0.0737	-0.0683	-0.0601
      | -0.0824	-0.0803	-0.0775	-0.0734	-0.0681	-0.0599
      | -0.082	-0.08	-0.0771	-0.073	-0.0677	-0.0596
      | -0.0816	-0.0795	-0.0767	-0.0726	-0.0673	-0.0592
      | -0.081	-0.079	-0.0761	-0.0721	-0.0668	-0.0587
      | -0.0804	-0.0783	-0.0755	-0.0715	-0.0663	-0.0582
      | -0.0796	-0.0776	-0.0748	-0.0708	-0.0656	-0.0577
      | -0.0788	-0.0768	-0.074	-0.0701	-0.0649	-0.057
      | -0.0779	-0.0759	-0.0732	-0.0693	-0.0642	-0.0563
      | ]
      ColumnIndex=|
      | [0.3	0.4	0.5	0.6	0.7	0.8
      | ]
  MYWX : Lookup2D  RowIndex=|  ColumnIndex=|  Table=|  SaturateOnIntegerOverflow=off  InputSameDT=off
      RowIndex=|
      | [-2
      | -1
      | 0.5
      | 1
      | 2
      | 3
      | 4
      | 5
      | 6
      | 7
      | 8
      | 9
      | 10
      | ]
      Table=|
      | [-0.0014 	-0.0013 	-0.0013 	-0.0012 	-0.0011 	-0.0010 
      | -0.0007 	-0.0007 	-0.0006 	-0.0006 	-0.0006 	-0.0005 
      | 0.0003 	0.0003 	0.0003 	0.0003 	0.0003 	0.0002 
      | 0.0007 	0.0007 	0.0006 	0.0006 	0.0006 	0.0005 
      | 0.0014 	0.0013 	0.0013 	0.0012 	0.0011 	0.0010 
      | 0.0020 	0.0020 	0.0019 	0.0018 	0.0017 	0.0015 
      | 0.0027 	0.0026 	0.0025 	0.0024 	0.0022 	0.0019 
      | 0.0033 	0.0032 	0.0031 	0.0030 	0.0027 	0.0024 
      | 0.0039 	0.0038 	0.0037 	0.0035 	0.0032 	0.0028 
      | 0.0045 	0.0044 	0.0042 	0.0040 	0.0037 	0.0033 
      | 0.0050 	0.0049 	0.0047 	0.0045 	0.0041 	0.0036 
      | 0.0055 	0.0054 	0.0052 	0.0049 	0.0046 	0.0040 
      | 0.0060 	0.0058 	0.0056 	0.0053 	0.0049 	0.0043 
      | ]
      ColumnIndex=|
      | [0.3	0.4	0.5	0.6	0.7	0.8
      | ]
  MYWY : Lookup2D  RowIndex=|  ColumnIndex=|  Table=|  SaturateOnIntegerOverflow=off  InputSameDT=off
      RowIndex=|
      | [-2
      | -1
      | 0.5
      | 1
      | 2
      | 3
      | 4
      | 5
      | 6
      | 7
      | 8
      | 9
      | 10
      | ]
      Table=|
      | [-0.0401	-0.039	-0.0377	-0.0357	-0.0331	-0.0291
      | -0.0403	-0.0393	-0.0379	-0.0359	-0.0333	-0.0293
      | -0.0407	-0.0397	-0.0383	-0.0363	-0.0337	-0.0296
      | -0.0408	-0.0398	-0.0384	-0.0364	-0.0337	-0.0297
      | -0.041	-0.04	-0.0386	-0.0366	-0.0339	-0.0298
      | -0.0412	-0.0402	-0.0387	-0.0367	-0.0341	-0.03
      | -0.0414	-0.0403	-0.0389	-0.0369	-0.0342	-0.0301
      | -0.0415	-0.0404	-0.039	-0.037	-0.0343	-0.0302
      | -0.0416	-0.0405	-0.0391	-0.037	-0.0344	-0.0303
      | -0.0416	-0.0406	-0.0392	-0.0371	-0.0344	-0.0303
      | -0.0417	-0.0406	-0.0392	-0.0371	-0.0345	-0.0303
      | -0.0417	-0.0406	-0.0392	-0.0371	-0.0345	-0.0303
      | -0.0417	-0.0406	-0.0392	-0.0371	-0.0344	-0.0303
      | ]
      ColumnIndex=|
      | [0.3	0.4	0.5	0.6	0.7	0.8
      | ]
  My : Outport
  wires:
  WX/1 -> Divide3/2
  WY/1 -> Divide2/2
  Beta/1 -> Divide1/2
  Ma/1 -> MYBETA/2, MYWY/2, MYWX/2
  alpha/1 -> MYBETA/1, MYWY/1, MYWX/1
  Add2/1 -> My/1
  Divide3/1 -> Add2/3
  Divide2/1 -> Add2/2
  MYWX/1 -> Divide3/1
  MYWY/1 -> Divide2/1
  MYBETA/1 -> Divide1/1
  Divide1/1 -> Add2/1

== system ASEToolBox/Aerocraft Model/ACE Equation of 6DOF's Motion/Aero Force & Moment/ACE Aerodynamic for 6DOF/Mz Subsystem ==
  Ma : Inport
  alpha : Inport  Port=2
  DeltZ : Inport  Port=3
  WZ : Inport  Port=4
  Add1 : Sum  Inputs=+++
  Divide2 : Product  Inputs=**
  Divide3 : Product  Inputs=**
  MZ0 : Lookup2D  RowIndex=[-2,-1,0.5,1,2,3,4,5,6,7,8,9,10]  ColumnIndex=[0.3,0.4,0.5,0.6,0.7,0.8]  Table=reshape([0.0795,0.0397,-0.0199,-0.0397,-0.0795,-0.1193,-0.1589,-0.1983,-0.2375,-0.2763,-0.3146,-0.3523,-0.3894,0.078,0.039,-0.0195,-0.039,-0.078,-0.117,-0.1558,-0.1945,-0.2329,-0.271,-0.3086,-0.3456,-0.382,0.0759,0.0379,-0.0189,-0.0379,-0.0759,-0.1138,-0.1516,-0.1892,-0.2266,-0.2637,-0.3003,-0.3364,-0.3718,0.0728,0.0364,-0.0182,-0.0364,-0.0728,-0.1092,-0.1455,-0.1816,-0.2175,-0.2531,-0.2883,-0.323,-0.3572,0.0687,0.0343,-0.0172,-0.0343,-0.0687,-0.1031,-0.1374,-0.1716,-0.2056,-0.2393,-0.2726,-0.3055,-0.3378,0.0624,0.0312,-0.0156,-0.0312,-0.0624,-0.0937,-0.1249,-0.1559,-0.1869,-0.2176,-0.248,-0.278,-0.3076],13,6)  SaturateOnIntegerOverflow=off  InputSameDT=off
  MZDeltZ : Lookup2D  RowIndex=|  ColumnIndex=|  Table=|  SaturateOnIntegerOverflow=off  InputSameDT=off
      RowIndex=|
      | [-2
      | -1
      | 0.5
      | 1
      | 2
      | 3
      | 4
      | 5
      | 6
      | 7
      | 8
      | 9
      | 10
      | ]
      Table=|
      | [0.0233	0.0237	0.0241	0.0246	0.0246	0.0246
      | 0.0233	0.0237	0.0242	0.0246	0.0246	0.0246
      | 0.0233	0.0237	0.0242	0.0246	0.0246	0.0246
      | 0.0233	0.0237	0.0242	0.0246	0.0246	0.0246
      | 0.0233	0.0237	0.0241	0.0246	0.0246	0.0246
      | 0.0232	0.0237	0.0241	0.0245	0.0245	0.0245
      | 0.0232	0.0236	0.024	0.0245	0.0245	0.0245
      | 0.0231	0.0235	0.024	0.0244	0.0244	0.0244
      | 0.023	0.0234	0.0239	0.0243	0.0243	0.0243
      | 0.0229	0.0233	0.0238	0.0242	0.0242	0.0242
      | 0.0228	0.0232	0.0236	0.0241	0.0241	0.0241
      | 0.0227	0.0231	0.0235	0.0239	0.0239	0.0239
      | 0.0225	0.0229	0.0233	0.0238	0.0238	0.0238
      | ]
      ColumnIndex=|
      | [0.3	0.4	0.5	0.6	0.7	0.8
      | ]
  MZWZ : Lookup2D  RowIndex=|  ColumnIndex=|  Table=|  SaturateOnIntegerOverflow=off  InputSameDT=off
      RowIndex=|
      | [-2
      | -1
      | 0.5
      | 1
      | 2
      | 3
      | 4
      | 5
      | 6
      | 7
      | 8
      | 9
      | 10
      | ]
      Table=|
      | [-0.0182	-0.0182	-0.0182	-0.0182	-0.0182	-0.0182
      | -0.0183	-0.0183	-0.0183	-0.0183	-0.0183	-0.0183
      | -0.0183	-0.0183	-0.0183	-0.0183	-0.0183	-0.0183
      | -0.0183	-0.0183	-0.0183	-0.0183	-0.0183	-0.0183
      | -0.0182	-0.0182	-0.0182	-0.0182	-0.0182	-0.0182
      | -0.0182	-0.0182	-0.0182	-0.0182	-0.0182	-0.0182
      | -0.0182	-0.0182	-0.0182	-0.0182	-0.0182	-0.0182
      | -0.0181	-0.0181	-0.0181	-0.0181	-0.0181	-0.0181
      | -0.018	-0.018	-0.018	-0.018	-0.018	-0.018
      | -0.018	-0.018	-0.018	-0.018	-0.018	-0.018
      | -0.0179	-0.0179	-0.0179	-0.0179	-0.0179	-0.0179
      | -0.0177	-0.0177	-0.0177	-0.0177	-0.0177	-0.0177
      | -0.0176	-0.0176	-0.0176	-0.0176	-0.0176	-0.0176
      | ]
      ColumnIndex=|
      | [0.3	0.4	0.5	0.6	0.7	0.8
      | ]
  Mz : Outport
  wires:
  DeltZ/1 -> Divide2/2
  MZDeltZ/1 -> Divide2/1
  WZ/1 -> Divide3/2
  Ma/1 -> MZ0/2, MZDeltZ/2, MZWZ/2
  alpha/1 -> MZ0/1, MZDeltZ/1, MZWZ/1
  MZWZ/1 -> Divide3/1
  Add1/1 -> Mz/1
  Divide3/1 -> Add1/3
  Divide2/1 -> Add1/2
  MZ0/1 -> Add1/1

== system ASEToolBox/Subsystem/Formation-Control/Consistent formation control /一致性控制——F1/Subsystem1 ==
  Constant : Constant  Value=0.01
  MATLAB Function : MATLAB Function  TreatAsAtomicUnit=on
  Mux : Mux  Inputs=3
  Ramp : simulink/Sources/Ramp  slope=1  start=0  InitialOutput=0
  wxyz : Outport
  wires:
  Ramp/1 -> MATLAB Function/1(i)
  Constant/1 -> MATLAB Function/2(dt)
  MATLAB Function/1(wx) -> Mux/1
  MATLAB Function/2(wy) -> Mux/3, Mux/2
  Mux/1 -> wxyz/1

== system ASEToolBox/Subsystem/Formation-Control/Consistent formation control /一致性控制——F2/Subsystem2 ==
  Constant : Constant  Value=0.01
  MATLAB Function : MATLAB Function  TreatAsAtomicUnit=on
  Mux : Mux  Inputs=3
  Ramp : simulink/Sources/Ramp  slope=1  start=0  InitialOutput=0
  wxyz : Outport
  wires:
  Ramp/1 -> MATLAB Function/1(i)
  Constant/1 -> MATLAB Function/2(dt)
  MATLAB Function/1(wx) -> Mux/1
  MATLAB Function/2(wy) -> Mux/3, Mux/2
  Mux/1 -> wxyz/1

== system ASEToolBox/Subsystem/Formation-Control/Consistent formation control /一致性控制——F3/Subsystem1 ==
  Constant : Constant  Value=0.01
  MATLAB Function : MATLAB Function  TreatAsAtomicUnit=on
  Mux : Mux  Inputs=3
  Ramp : simulink/Sources/Ramp  slope=1  start=0  InitialOutput=0
  wxyz : Outport
  wires:
  Ramp/1 -> MATLAB Function/1(i)
  Constant/1 -> MATLAB Function/2(dt)
  MATLAB Function/1(wx) -> Mux/1
  MATLAB Function/2(wy) -> Mux/3, Mux/2
  Mux/1 -> wxyz/1

== system ASEToolBox/Subsystem/Formation-Control/Follower1/Subsystem/get lmd ==
  Add : Sum  Inputs=+-
  Add1 : Sum  Inputs=+-
  Gain : Gain  Gain=0.707
  Gain1 : Gain  Gain=0.707
  Min : MinMax  Inputs=2
  lmd high : Constant  Value=lmd_high
  lmd low : Constant  Value=lmd_low
  v0_max : Constant  Value=v0_max
  v0_min : Constant  Value=v0_min
  lmd : Outport
  wires:
  v0_min/1 -> Add/1
  lmd low/1 -> Add/2
  Add/1 -> Gain/1
  v0_max/1 -> Add1/2
  lmd high/1 -> Add1/1
  Add1/1 -> Gain1/1
  Gain/1 -> Min/1
  Gain1/1 -> Min/2
  Min/1 -> lmd/1

== system ASEToolBox/Subsystem/Formation-Control/Follower2/Subsystem/get lmd ==
  Add : Sum  Inputs=+-
  Add1 : Sum  Inputs=+-
  Gain : Gain  Gain=0.707
  Gain1 : Gain  Gain=0.707
  Min : MinMax  Inputs=2
  lmd high : Constant  Value=6.45
  lmd low : Constant  Value=0.45
  v0_max : Constant  Value=3.5
  v0_min : Constant  Value=3
  lmd : Outport
  wires:
  Min/1 -> lmd/1
  Gain1/1 -> Min/2
  Gain/1 -> Min/1
  Add1/1 -> Gain1/1
  lmd high/1 -> Add1/1
  v0_max/1 -> Add1/2
  Add/1 -> Gain/1
  lmd low/1 -> Add/2
  v0_min/1 -> Add/1

== system ASEToolBox/Subsystem/Formation-Control/Follower3/Subsystem/get lmd ==
  Add : Sum  Inputs=+-
  Add1 : Sum  Inputs=+-
  Gain : Gain  Gain=0.707
  Gain1 : Gain  Gain=0.707
  Min : MinMax  Inputs=2
  lmd high : Constant  Value=6.45
  lmd low : Constant  Value=0.45
  v0_max : Constant  Value=3.5
  v0_min : Constant  Value=3
  lmd : Outport
  wires:
  v0_min/1 -> Add/1
  lmd low/1 -> Add/2
  Add/1 -> Gain/1
  v0_max/1 -> Add1/2
  lmd high/1 -> Add1/1
  Add1/1 -> Gain1/1
  Gain/1 -> Min/1
  Gain1/1 -> Min/2
  Min/1 -> lmd/1

== system ASEToolBox/Subsystem/GNC_EKF/Translation_estimate/V_Horizontal_estimation1/Integrator_V_Horizontal ==
  An : Inport
  dv : Inport  Port=2
  QGC_init : Inport  Port=3
  vn_gps : Inport  Port=4
  ve_gps : Inport  Port=5
  GPSenable : Inport  Port=6
  Delay : Delay  DelayLength=1  InitialConditionSource=Input port  ExternalReset=Rising
      settings: InputPortMap=u0,r5,p4
  Gain : Gain  Gain=0.8
  Gain2 : Gain  Gain=dt  SaturateOnIntegerOverflow=on  OutDataTypeStr=Inherit: Same as input  ParamDataTypeStr=Inherit: Same as input
  Mux : Mux  Inputs=2
  Product : Product
  Scope : Scope
      settings: ActiveDisplayYMinimum=-0.0503  ActiveDisplayYMaximum=0.05997  DataLoggingVariableName=ScopeData3
  Sum : Sum  Inputs=|++-
  V_n&e : Outport
  wires:
  GPSenable/1 -> Product/2
  dv/1 -> Product/1
  An/1 -> Gain2/1
  Gain2/1 -> Sum/1
  Sum/1 -> V_n&e/1, Delay/1
  QGC_init/1 -> Delay/2
  vn_gps/1 -> Mux/1
  ve_gps/1 -> Mux/2
  Mux/1 -> Delay/3
  Delay/1 -> Sum/2
  Product/1 -> Gain/1
  Gain/1 -> Scope/1, Sum/3

== system ASEToolBox/Subsystem/GNC_EKF/Translation_estimate/V_Horizontal_estimation1/Rxy_kalman filter1 ==
  X : Inport
  Z : Inport  Port=2
  Enable : Inport  Port=3
  Constant : Constant  Value=F  OutDataTypeStr=single
  Constant1 : Constant  Value=Q  OutDataTypeStr=single
  Constant2 : Constant  Value=R  OutDataTypeStr=single
  Constant3 : Constant  Value=P0  OutDataTypeStr=single
  Constant4 : Constant  Value=H  OutDataTypeStr=single
  Vxy kalman filter : Subsystem  TreatAsAtomicUnit=on
  XOut : Outport
  wires:
  Enable/1 -> Vxy kalman filter/9(Enable)
  Vxy kalman filter/1(XOut) -> XOut/1
  Constant1/1 -> Vxy kalman filter/5(Q)
  Constant4/1 -> Vxy kalman filter/4(H)
  Constant2/1 -> Vxy kalman filter/6(R)
  Constant3/1 -> Vxy kalman filter/8(P0)
  Z/1 -> Vxy kalman filter/1(Z)
  Constant/1 -> Vxy kalman filter/3(G), Vxy kalman filter/2(F)
  X/1 -> Vxy kalman filter/7(X)

== system ASEToolBox/Aerocraft Model/ACE Equation of 6DOF's Motion/ACE Rotation Motion/Attitude Dynamic /Omega_Tx1 Subsystem/Deal with zero ==
  In1 : Inport
  Constant : Constant  Value=0
  Constant1 : Constant  Value=0.001
  Relational Operator : RelationalOperator  Operator=~=
  Switch : Switch  Threshold=0.0001
  Out1 : Outport
  wires:
  In1/1 -> Switch/1, Relational Operator/1
  Switch/1 -> Out1/1
  Constant1/1 -> Switch/3
  Relational Operator/1 -> Switch/2
  Constant/1 -> Relational Operator/2

== system ASEToolBox/Aerocraft Model/ACE Equation of 6DOF's Motion/ACE Rotation Motion/Attitude Dynamic /Omega_Tx1 Subsystem1/Deal with zero ==
  In1 : Inport
  Constant : Constant  Value=0
  Constant1 : Constant  Value=0.000001
  Relational Operator : RelationalOperator  Operator=~=
  Switch : Switch  Threshold=0.0001
  Out1 : Outport
  wires:
  Constant/1 -> Relational Operator/2
  Relational Operator/1 -> Switch/2
  Constant1/1 -> Switch/3
  Switch/1 -> Out1/1
  In1/1 -> Switch/1, Relational Operator/1

== system ASEToolBox/Aerocraft Model/ACE Equation of 6DOF's Motion/ACE Rotation Motion/Attitude Dynamic /Omega_Tx1 Subsystem2/Deal with zero ==
  In1 : Inport
  Constant : Constant  Value=0
  Constant1 : Constant  Value=0.000001
  Relational Operator : RelationalOperator  Operator=~=
  Switch : Switch  Threshold=0.0001
  Out1 : Outport
  wires:
  In1/1 -> Relational Operator/1, Switch/1
  Switch/1 -> Out1/1
  Constant1/1 -> Switch/3
  Relational Operator/1 -> Switch/2
  Constant/1 -> Relational Operator/2

== system ASEToolBox/Aerocraft Model/ACE Equation of 6DOF's Motion/ACE Rotation Motion/calculate Eular 231/psi Subsystem/Deal with zero1 ==
  In1 : Inport
  Constant : Constant  Value=0
  Constant1 : Constant  Value=0.000001
  Relational Operator : RelationalOperator  Operator=~=
  Switch : Switch  Threshold=0.0001
  Out1 : Outport
  wires:
  Constant/1 -> Relational Operator/2
  Relational Operator/1 -> Switch/2
  Constant1/1 -> Switch/3
  Switch/1 -> Out1/1
  In1/1 -> Switch/1, Relational Operator/1

== system ASEToolBox/Subsystem/GNC_EKF/Translation_estimate/V_Horizontal_estimation1/Rxy_kalman filter1/Vxy kalman filter ==
  Z : Inport
  F : Inport  Port=2
  G : Inport  Port=3
  H : Inport  Port=4
  Q : Inport  Port=5
  R : Inport  Port=6
  X : Inport  Port=7
  P0 : Inport  Port=8
  Enable : Inport  Port=9
  Add1 : Sum
  Delay : Delay  DelayLength=1  InitialConditionSource=Input port
      settings: InputPortMap=u0,p4
  Gain4 : Gain  Gain=0.5
  Math Function : Math  Operator=transpose  SignedPower=on
  kalman : Subsystem
  XOut : Outport
  wires:
  P0/1 -> Delay/2
  Gain4/1 -> Delay/1
  Delay/1 -> kalman/7(P)
  Add1/1 -> Gain4/1
  Math Function/1 -> Add1/2
  Z/1 -> kalman/1(Z)
  F/1 -> kalman/2(F)
  G/1 -> kalman/3(G)
  H/1 -> kalman/4(H)
  Q/1 -> kalman/5(Q)
  R/1 -> kalman/6(R)
  X/1 -> kalman/8(X)
  kalman/1(POut) -> Math Function/1, Add1/1
  kalman/2(XOut) -> XOut/1
  Enable/1 -> kalman/9(Enable)

== system ASEToolBox/Subsystem/GNC_EKF/Translation_estimate/V_Horizontal_estimation1/Rxy_kalman filter1/Vxy kalman filter/kalman ==
  note: Xk/k-1=FXk-1
      | Xk=Xk/k-1+K(Z-h(Xk/k-1))
      | K=Pk/k-1H(HPk/k-1H+Rk)-1
      | Pk/k-1=FPk-1F+GQG
      | Pk=(I-KH)Pk/k-1
  Z : Inport
  F : Inport  Port=2
  G : Inport  Port=3
  H : Inport  Port=4
  Q : Inport  Port=5
  R : Inport  Port=6
  P : Inport  Port=7
  X : Inport  Port=8
  Enable : Inport  Port=9
  Scope : Scope  NumInputPorts=2
      settings: ActiveDisplayYMinimum=-1  ActiveDisplayYMaximum=1  DataLoggingVariableName=ScopeData2
  Subsystem : Subsystem
  Subsystem1 : Subsystem
  POut : Outport
  XOut : Outport  Port=2
  wires:
  X/1 -> [X]
  P/1 -> [P]
  Q/1 -> [Q]
  G/1 -> [G]
  F/1 -> [F]
  Z/1 -> [Z]
  [F] -> Subsystem/1(F)
  [G] -> Subsystem/2(G)
  [Q] -> Subsystem/3(Q)
  [X] -> Subsystem/4(X)
  [P] -> Subsystem/5(P)
  Subsystem/1(Xk_k_1) -> [Xk_k_1]
  Subsystem/2(Pk_k_1) -> [Pk_k_1]
  H/1 -> Subsystem1/3(H)
  R/1 -> Subsystem1/4(R)
  Subsystem1/1(POut) -> POut/1
  Subsystem1/2(XOut) -> XOut/1, Scope/2
  [Xk_k_1] -> Subsystem1/1(Xkk)
  [Pk_k_1] -> Subsystem1/2(Pkk)
  Enable/1 -> Subsystem1/Enable, Scope/1
  [Z] -> Subsystem1/5(Z)

== system ASEToolBox/Subsystem/GNC_EKF/Translation_estimate/V_Horizontal_estimation1/Rxy_kalman filter1/Vxy kalman filter/kalman/Subsystem ==
  F : Inport
  G : Inport  Port=2
  Q : Inport  Port=3
  X : Inport  Port=4
  P : Inport  Port=5
  Add : Sum
  Math Function3 : Math  Operator=transpose  SignedPower=on
  Math Function4 : Math  Operator=transpose  SignedPower=on
  MatrixMultiply : Product  Multiplication=Matrix(*)
  MatrixMultiply1 : Product  Inputs=3  Multiplication=Matrix(*)
  MatrixMultiply8 : Product  Inputs=3  Multiplication=Matrix(*)
  Xk_k_1 : Outport
  Pk_k_1 : Outport  Port=2
  wires:
  Math Function4/1 -> MatrixMultiply8/3
  [Q] -> MatrixMultiply8/2
  MatrixMultiply/1 -> [Xk_k_1]
  MatrixMultiply1/1 -> Add/1
  [F] -> Math Function3/1
  Math Function3/1 -> MatrixMultiply1/3
  [P] -> MatrixMultiply1/2
  [F] -> MatrixMultiply1/1
  Add/1 -> [Pk_k_1]
  [G] -> MatrixMultiply8/1
  MatrixMultiply8/1 -> Add/2
  [X] -> MatrixMultiply/2
  [G] -> Math Function4/1
  [F] -> MatrixMultiply/1
  F/1 -> [F]
  G/1 -> [G]
  Q/1 -> [Q]
  X/1 -> [X]
  P/1 -> [P]
  [Xk_k_1] -> Xk_k_1/1
  [Pk_k_1] -> Pk_k_1/1
